simulink model "single_PID_actual"  (R2024b)
settings: Solver=VariableStepAuto  StartTime=0.001  StopTime=4  FixedStep=0.0001  RelTol=1e-3
undefined symbols (not defined in the file or in its folder): DiscIntNeverNeededParam
libraries: simulink x2
settings Model: Creator=kentliukx  LastModifiedBy=kentliukx

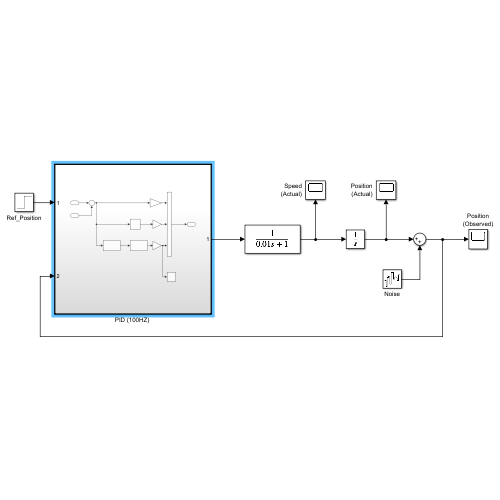
[thumbnail: Simulink's stored preview of the top-level diagram]
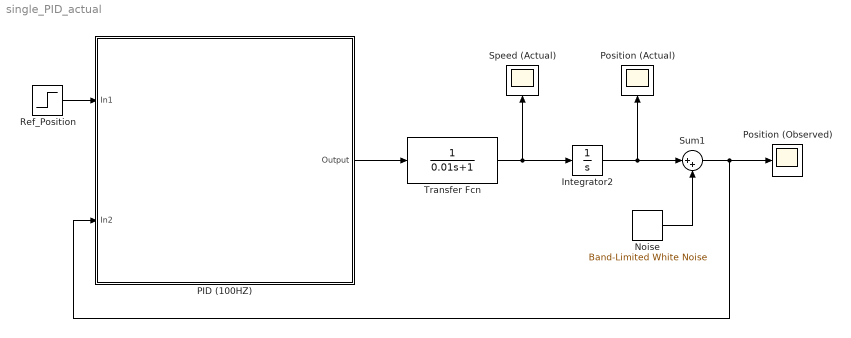
== system single_PID_actual ==
  Integrator2 : Integrator
  Noise : simulink/Sources/Band-Limited White Noise  Cov=[0.00001]  Ts=0.001  seed=[23341]
  "PID (100HZ) " : Subsystem  TreatAsAtomicUnit=on  SystemSampleTime=0.01
  Position (Actual) : Scope
  Position (Observed) : Scope
  Ref_Position : Step  SampleTime=0
  Speed (Actual) : Scope
  Sum1 : Sum  Inputs=|++
  Transfer Fcn : TransferFcn  Denominator=[0.01 1]
  wires:
  Transfer Fcn/1 -> Integrator2/1, Speed (Actual)/1
  Integrator2/1 -> Sum1/1, Position (Actual)/1
  Noise/1 -> Sum1/2
  "PID (100HZ) "/1(Output) -> Transfer Fcn/1
  Sum1/1 -> Position (Observed)/1, "PID (100HZ) "/2(In2)
  Ref_Position/1 -> "PID (100HZ) "/1(In1)

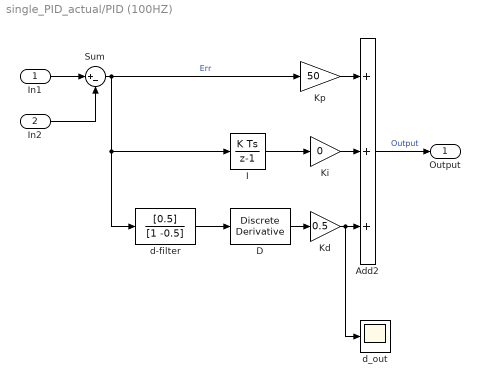
== system single_PID_actual/PID (100HZ)  ==
  In1 : Inport
  In2 : Inport  Port=2
  Add2 : Sum  Inputs=+++
  D : simulink/Discrete/Discrete Derivative  gainval=1.0  ICPrevScaledInput=0.0  OutMin=[]  OutMax=[]  OutDataType=fixdt(1, 16)  OutScaling=2^-10  DoSatur=off
  I : DiscreteIntegrator  SampleTime=-1  ICPrevOutput=DiscIntNeverNeededParam  ICPrevScaledInput=DiscIntNeverNeededParam
  Kd : Gain  Gain=0.5
  Ki : Gain  Gain=0
  Kp : Gain  Gain=50
  Sum : Sum  Inputs=|+-
  d-filter : DiscreteFilter  Numerator=[0.5]  Denominator=[1 -0.5]
  d_out : Scope
  Output : Outport
  wires:
  Sum/1 -> Kp/1, d-filter/1, I/1  "Err"
  D/1 -> Kd/1
  Ki/1 -> Add2/2
  Kp/1 -> Add2/1
  In2/1 -> Sum/2
  Add2/1 -> Output/1  "Output"
  In1/1 -> Sum/1
  I/1 -> Ki/1
  d-filter/1 -> D/1
  Kd/1 -> d_out/1, Add2/3
